simulink subsystem "hour_day_season"  (R2025b)
settings: Solver=VariableStepAuto  StartTime=0.0  StopTime=10.0  RelTol=1e-3
settings Model: Creator=lenovo  LastModifiedBy=lenovo

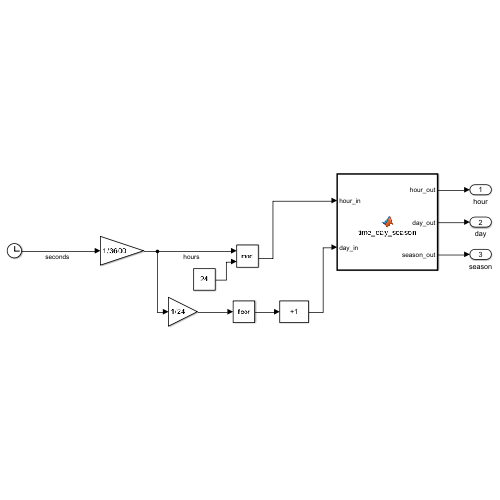
[thumbnail: Simulink's stored preview of the top-level diagram]
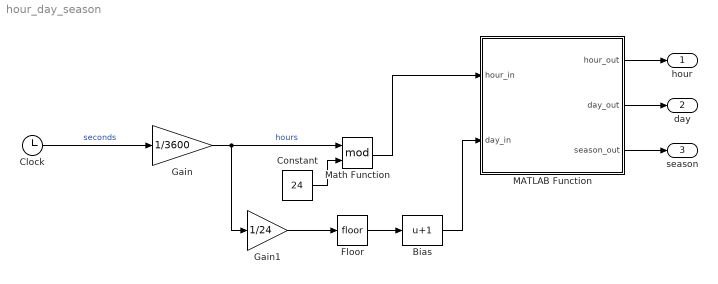
== system hour_day_season ==
  Bias : Bias  Bias=1  SaturateOnIntegerOverflow=off
  Clock : Clock
  Constant : Constant  Value=24
  Floor : Rounding
  Gain : Gain  Gain=1/3600
  Gain1 : Gain  Gain=1/24
  MATLAB Function : MATLAB Function  TreatAsAtomicUnit=on
  Math Function : Math  Operator=mod
  hour : Outport
  day : Outport  Port=2
  season : Outport  Port=3
  wires:
  Clock/1 -> Gain/1  "seconds"
  Gain/1 -> Gain1/1, Math Function/1  "hours"
  Constant/1 -> Math Function/2
  Math Function/1 -> MATLAB Function/1(hour_in)
  Gain1/1 -> Floor/1
  Floor/1 -> Bias/1
  Bias/1 -> MATLAB Function/2(day_in)
  MATLAB Function/1(hour_out) -> hour/1
  MATLAB Function/2(day_out) -> day/1
  MATLAB Function/3(season_out) -> season/1

== matlab function hour_day_season/MATLAB Function ==
  data: hour_in input; hour_out output; day_in input; day_out output; season_out output
function [hour_out, day_out, season_out] = time_day_season(hour_in, day_in)

% Pass through signals
hour_out = hour_in;
day_out  = day_in;

% Season changes with day progression
% Define cycle length (e.g., 90 days per season)
cycle_day = mod(day_in, 270);  % 3 seasons × 90 days

if cycle_day < 90
    season_out = 1;   % Summer
elseif cycle_day < 180
    season_out = 2;   % Rainy
else
    season_out = 3;   % Winter
end

end
